simulink model "FullFMS_2026_02_18_V0_3_9"  (R2025b)
settings: Solver=ode23tb  StartTime=0.0  StopTime=inf  MaxStep=0.1  RelTol=1e-2
PreLoadFcn:
  | load("BUS_CONFIG.mat")
libraries: opcualib x8
(part 4 of 4)

== matlab function FullFMS_2026_02_18_V0_3_9/MATLAB Function ==
  data: u1 input; C_24_CRoute_In output; u2 input; u3 input; u4 input; u5 input; u6 input; u7 input; u8 input; u9 input; u10 input; u11 input; u12 input; u13 input; u14 input; u15 input; u16 input; u17 input; u18 input; u19 input; u20 input; u21 input; u22 input; u23 input; u24 input; u25 input; u26 input; u27 input; u28 input; u29 input; u30 input; u31 input; u32 input; u33 input; u34 input; u35 input; u36 input; u37 input; u38 input; u39 input; u40 input; u41 input; u42 input; u43 input; u44 input; u45 input; u46 input; u47 input; u48 input; u49 input; u50 input; u51 input; u52 input; u53 input; u54 input; u55 input; u56 input; u57 input; u58 input; u59 input; u60 input; u61 input; u62 input; u63 input; u64 input; u65 input; u66 input; C_25_CRoute_In output; C_26_CRoute_In output; C_27_CRoute_In output; C_28_CRoute_In output; C_29_CRoute_In output; C_24_Request output; C_24_CartDel output; C_24_CRoute_Out output; C_25_Request output; C_25_CartDel output; C_25_CRoute_Out output; C_26_Request output; C_26_CartDel output; C_26_CRoute_Out output; C_27_Request output; C_27_CartDel output; C_27_CRoute_Out output; C_28_Request output; C_28_CartDel output; C_28_CRoute_Out output; C_29_Request output; C_29_CartDel output; C_29_CRoute_Out output; F_22_Led_On output; F_22_Led_Off output; F_22_Conveyor output; F_24_Release_FB output; F_25_Release_FB output; F_26_Release_FB output; F_27_Release_FB output; F_28_Release_FB output; F_29_Release_FB output; O_20_On output; O_20_Off output; O_20_Controler_On output; O_24_Cart_Stat output; O_24_Cart_Next output; O_24_Optic output; O_24_Count output; O_24_Pist_Bck output; O_25_Cart_Stat output; O_25_Cart_Next output; O_25_Optic output; O_25_Count output; O_25_Pist_Back output; O_26_Cart_Stat output; O_26_Cart_Next output; O_26_Optic output; O_26_Count output; O_26_Pist_Back output; O_27_Cart_Stat output; O_27_Cart_Next output; O_27_Optic output; O_27_Count output; O_27_Pist_Back output; O_28_Cart_Stat output; O_28_Cart_Next output; O_28_Optic output; O_28_Count output; O_28_Pist_Back output; O_29_Cart_Stat output; O_29_Cart_Next output; O_29_Optic output; O_29_Count output; O_29_Pist_Back output
function [C_24_CRoute_In, C_25_CRoute_In, C_26_CRoute_In, C_27_CRoute_In, ...
    C_28_CRoute_In, C_29_CRoute_In, C_24_Request, C_24_CartDel, C_24_CRoute_Out, ...
    C_25_Request, C_25_CartDel, C_25_CRoute_Out, C_26_Request, C_26_CartDel, ...
    C_26_CRoute_Out, C_27_Request, C_27_CartDel, C_27_CRoute_Out, C_28_Request, ...
    C_28_CartDel, C_28_CRoute_Out, C_29_Request, C_29_CartDel, C_29_CRoute_Out, ...
    F_22_Led_On, F_22_Led_Off, F_22_Conveyor, F_24_Release_FB, F_25_Release_FB, ...
    F_26_Release_FB, F_27_Release_FB, F_28_Release_FB, F_29_Release_FB, ...
    O_20_On, O_20_Off, O_20_Controler_On, O_24_Cart_Stat, O_24_Cart_Next, ...
    O_24_Optic, O_24_Count, O_24_Pist_Bck, O_25_Cart_Stat, O_25_Cart_Next, ...
    O_25_Optic, O_25_Count, O_25_Pist_Back, O_26_Cart_Stat, O_26_Cart_Next, ...
    O_26_Optic, O_26_Count, O_26_Pist_Back, O_27_Cart_Stat, O_27_Cart_Next, ...
    O_27_Optic, O_27_Count, O_27_Pist_Back, O_28_Cart_Stat, O_28_Cart_Next, ...
    O_28_Optic, O_28_Count, O_28_Pist_Back, O_29_Cart_Stat, O_29_Cart_Next, ...
    O_29_Optic, O_29_Count, O_29_Pist_Back] = fcn_MASTER(u1, u2, u3, u4, u5, u6, u7, u8, u9, u10, u11, u12, u13, u14, u15, u16, u17, u18, u19, u20, u21, u22, u23, u24, u25, u26, u27, u28, u29, u30, u31, u32, u33, u34, u35, u36, u37, u38, u39, u40, u41, u42, u43, u44, u45, u46, u47, u48, u49, u50, u51, u52, u53, u54, u55, u56, u57, u58, u59, u60, u61, u62, u63, u64, u65, u66)

% Primeiro bloco - Controle (24 entradas)
C_24_CRoute_In = u1;
C_25_CRoute_In = u2;
C_26_CRoute_In = u3;
C_27_CRoute_In = u4;
C_28_CRoute_In = u5;
C_29_CRoute_In = u6;
C_24_Request = u7;
C_24_CartDel = u8;
C_24_CRoute_Out = u9;
C_25_Request = u10;
C_25_CartDel = u11;
C_25_CRoute_Out = u12;
C_26_Request = u13;
C_26_CartDel = u14;
C_26_CRoute_Out = u15;
C_27_Request = u16;
C_27_CartDel = u17;
C_27_CRoute_Out = u18;
C_28_Request = u19;
C_28_CartDel = u20;
C_28_CRoute_Out = u21;
C_29_Request = u22;
C_29_CartDel = u23;
C_29_CRoute_Out = u24;

% Segundo bloco - Feedback (9 entradas, começando em u25)
F_22_Led_On = u25;
F_22_Led_Off = u26;
F_22_Conveyor = u27;
F_24_Release_FB = u28;
F_25_Release_FB = u29;
F_26_Release_FB = u30;
F_27_Release_FB = u31;
F_28_Release_FB = u32;
F_29_Release_FB = u33;

% Terceiro bloco - Sensores (33 entradas, começando em u34)
O_20_On = u34;
O_20_Off = u35;
O_20_Controler_On = u36;
O_24_Cart_Stat = u37;
O_24_Cart_Next = u38;
O_24_Optic = u39;
O_24_Count = u40;
O_24_Pist_Bck = u41;
O_25_Cart_Stat = u42;
O_25_Cart_Next = u43;
O_25_Optic = u44;
O_25_Count = u45;
O_25_Pist_Back = u46;
O_26_Cart_Stat = u47;
O_26_Cart_Next = u48;
O_26_Optic = u49;
O_26_Count = u50;
O_26_Pist_Back = u51;
O_27_Cart_Stat = u52;
O_27_Cart_Next = u53;
O_27_Optic = u54;
O_27_Count = u55;
O_27_Pist_Back = u56;
O_28_Cart_Stat = u57;
O_28_Cart_Next = u58;
O_28_Optic = u59;
O_28_Count = u60;
O_28_Pist_Back = u61;
O_29_Cart_Stat = u62;
O_29_Cart_Next = u63;
O_29_Optic = u64;
O_29_Count = u65;
O_29_Pist_Back = u66;

end

== matlab function FullFMS_2026_02_18_V0_3_9/MATLAB Function1 ==
  data: u1 input; A_34_Request output; u2 input; u3 input; u4 input; u5 input; u6 input; u7 input; u8 input; u9 input; u10 input; u11 input; u12 input; u13 input; u14 input; u15 input; u16 input; u17 input; u18 input; u19 input; u20 input; u21 input; u22 input; u23 input; u24 input; u25 input; u26 input; u27 input; u28 input; u29 input; u30 input; u31 input; u32 input; u33 input; u34 input; u35 input; u36 input; u37 input; u38 input; u39 input; u40 input; u41 input; u42 input; u43 input; u44 input; u45 input; u46 input; u47 input; u48 input; u49 input; u50 input; u51 input; u52 input; u53 input; u54 input; u55 input; u56 input; u57 input; u58 input; u59 input; u60 input; u61 input; u62 input; u63 input; u64 input; u65 input; u66 input; A_34_No_Cart output; A_34_Cart_Full output; A_34_CRoute_Out output; A_32_RoboCartID output; A_34_Cart_Stat output; A_34_Cart_Next output; A_34_Optic output; A_34_Count output; A_34_Pist_Bck output; A_34_Release_FB output; A_34_CRoute_In output; C_30_Robot1 output; C_30_Robot2 output; C_35_Part_Del output; F_33_Led_Start output; F_33_Led_Reset output; F_33_Led_Extra1 output; F_33_Led_Extra2 output; F_33_Spring_Cyl output; F_33_Cover_Cyl output; O_31_Start output; O_31_Stop output; O_31_Reset output; O_31_Part_in_Claw output; O_31_Orientation output; O_32_Sp_Cyl_Bck output; O_32_Sp_Cyl_Fwd output; O_32_Co_Cyl_Bck output; O_32_Co_Cyl_Fwd output; O_32_Sp_PickUp output; O_32_Co_PickUp output; O_32_CoMag_Empty output; A_44_Request output; A_44_No_Cart output; A_44_Cart_Full output; A_44_CRoute_In output; A_43_StorCartID output; A_44_Cart_Stat output; A_44_Cart_Next output; A_44_Optic output; A_44_Count output; A_44_Pist_Bck output; A_44_Release_FB output; A_44_CRoute_Out output; C_45_Initialization output; C_42_Profibus output; C_45_Start output; C_45_StorePart output; C_45_RetrievePart output; F_43_Led_Start output; F_43_Led_Reset output; F_43_Led_Extra1 output; F_43_Led_Extra2 output; F_43_Panel_O4 output; F_43_Panel_O5 output; F_43_Panel_O6 output; F_43_Panel_O7 output; O_41_Start output; O_41_Stop output; O_41_Key_Pos output; O_41_Reset output; O_41_Panel_I4 output; O_41_Panel_I5 output; O_41_Panel_I6 output; O_41_Panel_I7 output
function [A_34_Request, A_34_No_Cart, A_34_Cart_Full, A_34_CRoute_Out, ...
    A_32_RoboCartID, A_34_Cart_Stat, A_34_Cart_Next, A_34_Optic, A_34_Count, ...
    A_34_Pist_Bck, A_34_Release_FB, A_34_CRoute_In, C_30_Robot1, C_30_Robot2,...
    C_35_Part_Del,F_33_Led_Start, F_33_Led_Reset, F_33_Led_Extra1, F_33_Led_Extra2, ...
    F_33_Spring_Cyl, F_33_Cover_Cyl, ...
    O_31_Start, O_31_Stop, O_31_Reset, O_31_Part_in_Claw, O_31_Orientation, ...
    O_32_Sp_Cyl_Bck, O_32_Sp_Cyl_Fwd, O_32_Co_Cyl_Bck, O_32_Co_Cyl_Fwd, ...
    O_32_Sp_PickUp, O_32_Co_PickUp, O_32_CoMag_Empty, ...
    A_44_Request, A_44_No_Cart, A_44_Cart_Full, A_44_CRoute_In, ...
    A_43_StorCartID, A_44_Cart_Stat, A_44_Cart_Next, A_44_Optic, A_44_Count, ...
    A_44_Pist_Bck, A_44_Release_FB, A_44_CRoute_Out, ...
    C_45_Initialization, C_42_Profibus, C_45_Start, C_45_StorePart, ...
    C_45_RetrievePart, ...
    F_43_Led_Start, F_43_Led_Reset, F_43_Led_Extra1, F_43_Led_Extra2, ...
    F_43_Panel_O4, F_43_Panel_O5, F_43_Panel_O6, F_43_Panel_O7, ...
    O_41_Start, O_41_Stop, O_41_Key_Pos, O_41_Reset, O_41_Panel_I4, ...
    O_41_Panel_I5, O_41_Panel_I6, O_41_Panel_I7] = ...
    fcn_ROBOT_STORAGE(u1, u2, u3, u4, u5, u6, u7, u8, u9, u10, u11, u12, ...
    u13, u14, u15, u16, u17, u18, u19, u20, u21, u22, u23, u24, u25, u26, ...
    u27, u28, u29, u30, u31, u32, u33, u34, u35, u36, u37, u38, u39, u40, ...
    u41, u42, u43, u44, u45, u46, u47, u48, u49, u50, u51, u52, u53, u54, ...
    u55, u56, u57, u58, u59, u60, u61, u62, u63, u64, u65, u66)

% Primeiro bloco - Asi (12 entradas: u1-u12)
A_34_Request = u1;
A_34_No_Cart = u2;
A_34_Cart_Full = u3;
A_34_CRoute_Out = u4;
A_32_RoboCartID = u5;
A_34_Cart_Stat = u6;
A_34_Cart_Next = u7;
A_34_Optic = u8;
A_34_Count = u9;
A_34_Pist_Bck = u10;
A_34_Release_FB = u11;
A_34_CRoute_In = u12;

% Segundo bloco - Control (3 entradas: u13-u15)
C_30_Robot1 = u13;
C_30_Robot2 = u14;
C_35_Part_Del = u15;

% Terceiro bloco - Feedback (6 entradas: u16-u21)
F_33_Led_Start = u16;
F_33_Led_Reset = u17;
F_33_Led_Extra1 = u18;
F_33_Led_Extra2 = u19;
F_33_Spring_Cyl = u20;
F_33_Cover_Cyl = u21;

% Quarto bloco - Sensors (12 entradas: u22-u33)
O_31_Start = u22;
O_31_Stop = u23;
O_31_Reset = u24;
O_31_Part_in_Claw = u25;
O_31_Orientation = u26;
O_32_Sp_Cyl_Bck = u27;
O_32_Sp_Cyl_Fwd = u28;
O_32_Co_Cyl_Bck = u29;
O_32_Co_Cyl_Fwd = u30;
O_32_Sp_PickUp = u31;
O_32_Co_PickUp = u32;
O_32_CoMag_Empty = u33;

% Quinto bloco - Asi_store (12 entradas: u34-u45)
A_44_Request = u34;
A_44_No_Cart = u35;
A_44_Cart_Full = u36;
A_44_CRoute_In = u37;
A_43_StorCartID = u38;
A_44_Cart_Stat = u39;
A_44_Cart_Next = u40;
A_44_Optic = u41;
A_44_Count = u42;
A_44_Pist_Bck = u43;
A_44_Release_FB = u44;
A_44_CRoute_Out = u45;

% Sexto bloco - Control_Storage (5 entradas: u46-u50)
C_45_Initialization = u46;
C_42_Profibus = u47;
C_45_Start = u48;
C_45_StorePart = u49;
C_45_RetrievePart = u50;

% Sétimo bloco - Feedback_storage (8 entradas: u51-u58)
F_43_Led_Start = u51;
F_43_Led_Reset = u52;
F_43_Led_Extra1 = u53;
F_43_Led_Extra2 = u54;
F_43_Panel_O4 = u55;
F_43_Panel_O5 = u56;
F_43_Panel_O6 = u57;
F_43_Panel_O7 = u58;

% Oitavo bloco - Sensors_40 (8 entradas: u59-u66)
O_41_Start = u59;
O_41_Stop = u60;
O_41_Key_Pos = u61;
O_41_Reset = u62;
O_41_Panel_I4 = u63;
O_41_Panel_I5 = u64;
O_41_Panel_I6 = u65;
O_41_Panel_I7 = u66;
end

== matlab function FullFMS_2026_02_18_V0_3_9/MATLAB Function2 ==
  data: u1 input; A_54_Request output; u2 input; u3 input; u4 input; u5 input; u6 input; u7 input; u8 input; u9 input; u10 input; u11 input; u12 input; u13 input; u14 input; u15 input; u16 input; u17 input; u18 input; u19 input; u20 input; u21 input; u22 input; u23 input; u24 input; u25 input; u26 input; u27 input; u28 input; u29 input; u30 input; u31 input; u32 input; u33 input; u34 input; u35 input; u36 input; u37 input; u38 input; u39 input; u40 input; u41 input; u42 input; u43 input; u44 input; A_54_No_Cart output; A_54_Cart_Full output; A_54_CRoute_Out output; A_53_SortCartID output; A_54_Cart_Stat output; A_54_Cart_Next output; A_54_Optic output; A_54_Count output; A_54_Pist_Bck output; A_54_Release_FB output; A_54_CRoute_In output; C_55_Initialization output; C_55_PD_Sort output; C_52_Profibus output; C_55_Start output; C_55_Cart2Del output; F_52_Claw_2_Del output; F_52_Claw_2_Cart output; F_52_Claw_Down output; F_52_Close_Claw output; F_53_Led_Start output; F_53_Led_Reset output; F_53_Led_Extra1 output; F_53_Led_Extra2 output; F_53_Panel_O4 output; F_53_Panel_O5 output; F_53_Panel_O6 output; F_53_Panel_O7 output; O_50_Part_Reserve output; O_50_Claw_Cart output; O_50_Claw_Del output; O_50_Claw_Reserve output; O_50_Claw_Low output; O_50_Claw_High output; O_50_Part_in_Claw output; O_51_Start output; O_51_Stop output; O_51_Key_Pos output; O_51_Reset output; O_51_Panel_I4 output; O_51_Panel_I5 output; O_51_Panel_I6 output; O_51_Panel_I7 output
function [A_54_Request, A_54_No_Cart, A_54_Cart_Full, A_54_CRoute_Out, ...
    A_53_SortCartID, A_54_Cart_Stat, A_54_Cart_Next, A_54_Optic, A_54_Count, ...
    A_54_Pist_Bck, A_54_Release_FB, A_54_CRoute_In, ...
    C_55_Initialization, C_55_PD_Sort, C_52_Profibus, C_55_Start, C_55_Cart2Del, ...
    F_52_Claw_2_Del, F_52_Claw_2_Cart, F_52_Claw_Down, F_52_Close_Claw, ...
    F_53_Led_Start, F_53_Led_Reset, F_53_Led_Extra1, F_53_Led_Extra2, ...
    F_53_Panel_O4, F_53_Panel_O5, F_53_Panel_O6, F_53_Panel_O7, ...
    O_50_Part_Reserve, O_50_Claw_Cart, O_50_Claw_Del, O_50_Claw_Reserve, ...
    O_50_Claw_Low, O_50_Claw_High, O_50_Part_in_Claw, O_51_Start, O_51_Stop, ...
    O_51_Key_Pos, O_51_Reset, O_51_Panel_I4, O_51_Panel_I5, O_51_Panel_I6, ...
    O_51_Panel_I7] = ...
    fcn_HD1(u1, u2, u3, u4, u5, u6, u7, u8, u9, u10, u11, u12, ...
    u13, u14, u15, u16, u17, u18, u19, u20, u21, u22, u23, u24, u25, u26, ...
    u27, u28, u29, u30, u31, u32, u33, u34, u35, u36, u37, u38, u39, u40, ...
    u41, u42, u43, u44)

% Primeiro bloco - Asi (12 entradas: u1-u12)
A_54_Request = u1;
A_54_No_Cart = u2;
A_54_Cart_Full = u3;
A_54_CRoute_Out = u4;
A_53_SortCartID = u5;
A_54_Cart_Stat = u6;
A_54_Cart_Next = u7;
A_54_Optic = u8;
A_54_Count = u9;
A_54_Pist_Bck = u10;
A_54_Release_FB = u11;
A_54_CRoute_In = u12;

% Segundo bloco - Control (5 entradas: u13-u17)
C_55_Initialization = u13;
C_55_PD_Sort = u14;
C_52_Profibus = u15;
C_55_Start = u16;
C_55_Cart2Del = u17;

% Terceiro bloco - Feedback (12 entradas: u18-u29)
F_52_Claw_2_Del = u18;
F_52_Claw_2_Cart = u19;
F_52_Claw_Down = u20;
F_52_Close_Claw = u21;
F_53_Led_Start = u22;
F_53_Led_Reset = u23;
F_53_Led_Extra1 = u24;
F_53_Led_Extra2 = u25;
F_53_Panel_O4 = u26;
F_53_Panel_O5 = u27;
F_53_Panel_O6 = u28;
F_53_Panel_O7 = u29;

% Quarto bloco - Sensors (15 entradas: u30-u44)
O_50_Part_Reserve = u30;
O_50_Claw_Cart = u31;
O_50_Claw_Del = u32;
O_50_Claw_Reserve = u33;
O_50_Claw_Low = u34;
O_50_Claw_High = u35;
O_50_Part_in_Claw = u36;
O_51_Start = u37;
O_51_Stop = u38;
O_51_Key_Pos = u39;
O_51_Reset = u40;
O_51_Panel_I4 = u41;
O_51_Panel_I5 = u42;
O_51_Panel_I6 = u43;
O_51_Panel_I7 = u44;

end

== matlab function FullFMS_2026_02_18_V0_3_9/MATLAB Function3 ==
  data: u1 input; C_65_Initialization output; u2 input; u3 input; u4 input; u5 input; u6 input; u7 input; u8 input; u9 input; u10 input; u11 input; u12 input; u13 input; u14 input; u15 input; u16 input; u17 input; u18 input; u19 input; u20 input; u21 input; u22 input; u23 input; u24 input; u25 input; u26 input; u27 input; u28 input; u29 input; u30 input; u31 input; u32 input; u33 input; u34 input; u35 input; u36 input; u37 input; u38 input; u39 input; C_65_ID_1 output; C_65_ID_2 output; C_65_Part_Sorted output; C_62_Profibus output; C_65_RBS_Output output; C_65_RSB_Output output; C_65_BRS_Output output; C_65_BSR_Output output; C_65_SRB_Output output; C_65_SBR_Output output; F_62_Conveyor output; F_62_P1 output; F_62_P2 output; F_62_Identify output; F_63_Led_Start output; F_63_Led_Reset output; F_63_Led_Extra1 output; F_63_Led_Extra2 output; F_63_Panel_O4 output; F_63_Panel_O5 output; F_63_Panel_O6 output; F_63_Panel_O7 output; O_60_SPart output; O_60_Slnd output; O_60_SPhoto output; O_60_Part_Pass output; O_60_SL1_Bck output; O_60_SL1_Fwd output; O_60_SL2_Bck output; O_60_SL2_Fwd output; O_61_Start output; O_61_Stop output; O_61_Key_Pos output; O_61_Reset output; O_61_Panel_I4 output; O_61_Panel_I5 output; O_61_Panel_I6 output; O_61_Panel_I7 output
function [C_65_Initialization, C_65_ID_1, C_65_ID_2, C_65_Part_Sorted, ...
    C_62_Profibus, C_65_RBS_Output, C_65_RSB_Output, C_65_BRS_Output, ...
    C_65_BSR_Output, C_65_SRB_Output, C_65_SBR_Output, ...
    F_62_Conveyor, F_62_P1, F_62_P2, F_62_Identify, ...
    F_63_Led_Start, F_63_Led_Reset, F_63_Led_Extra1, F_63_Led_Extra2, ...
    F_63_Panel_O4, F_63_Panel_O5, F_63_Panel_O6, F_63_Panel_O7, ...
    O_60_SPart, O_60_Slnd, O_60_SPhoto, O_60_Part_Pass, ...
    O_60_SL1_Bck, O_60_SL1_Fwd, O_60_SL2_Bck, O_60_SL2_Fwd, ...
    O_61_Start, O_61_Stop, O_61_Key_Pos, O_61_Reset, ...
    O_61_Panel_I4, O_61_Panel_I5, O_61_Panel_I6, O_61_Panel_I7] = ...
    fcn_SORT(u1, u2, u3, u4, u5, u6, u7, u8, u9, u10, u11, ...
    u12, u13, u14, u15, u16, u17, u18, u19, u20, u21, u22, u23, u24, u25, ...
    u26, u27, u28, u29, u30, u31, u32, u33, u34, u35, u36, u37, u38, u39)

% Primeiro bloco - Control (11 entradas: u1-u11)
C_65_Initialization = u1;
C_65_ID_1           = u2;
C_65_ID_2           = u3;
C_65_Part_Sorted    = u4;
C_62_Profibus       = u5;
C_65_RBS_Output     = u6;
C_65_RSB_Output     = u7;
C_65_BRS_Output     = u8;
C_65_BSR_Output     = u9;
C_65_SRB_Output     = u10;
C_65_SBR_Output     = u11;

% Segundo bloco - Feedback (12 entradas: u12-u23)
F_62_Conveyor   = u12;
F_62_P1         = u13;
F_62_P2         = u14;
F_62_Identify   = u15;
F_63_Led_Start  = u16;
F_63_Led_Reset  = u17;
F_63_Led_Extra1 = u18;
F_63_Led_Extra2 = u19;
F_63_Panel_O4   = u20;
F_63_Panel_O5   = u21;
F_63_Panel_O6   = u22;
F_63_Panel_O7   = u23;

% Terceiro bloco - Sensors (16 entradas: u24-u39)
O_60_SPart      = u24;
O_60_Slnd       = u25;
O_60_SPhoto     = u26;
O_60_Part_Pass  = u27;
O_60_SL1_Bck    = u28;
O_60_SL1_Fwd    = u29;
O_60_SL2_Bck    = u30;
O_60_SL2_Fwd    = u31;
O_61_Start      = u32;
O_61_Stop       = u33;
O_61_Key_Pos    = u34;
O_61_Reset      = u35;
O_61_Panel_I4   = u36;
O_61_Panel_I5   = u37;
O_61_Panel_I6   = u38;
O_61_Panel_I7   = u39;

end
